simulink model "B2_AutoHeadlamp"  (R2022b)
settings: Solver=FixedStepDiscrete  StartTime=0.0  StopTime=45  FixedStep=Ts  RelTol=1e-3
values from neighbouring files (symbols this model uses):
  LUX_OFF = 2000    [build_B2_AutoHeadlamp.m]
  LUX_ON = 1000    [build_B2_AutoHeadlamp.m]
  T_OFF = 5    [build_B2_AutoHeadlamp.m]
  T_ON = 2    [build_B2_AutoHeadlamp.m]
  T_TUNNEL = 0.3    [build_B2_AutoHeadlamp.m]
  Ts = 0.01    [build_B2_AutoHeadlamp.m]    (also in build_B3_AHB.m)
settings Model: Creator=LENOVO  LastModifiedBy=LENOVO

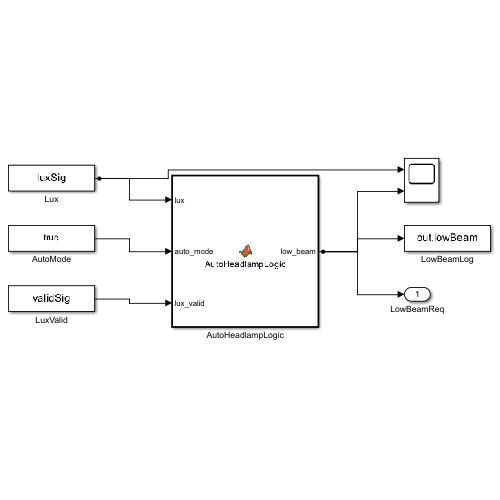
[thumbnail: Simulink's stored preview of the top-level diagram]
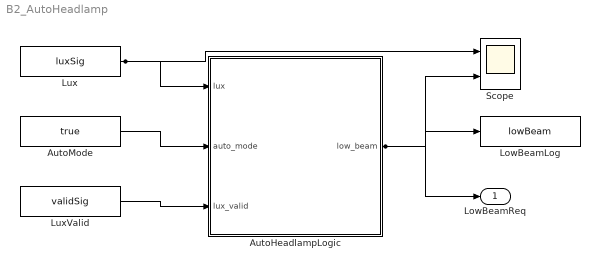
== system B2_AutoHeadlamp ==
  AutoHeadlampLogic : MATLAB Function  TreatAsAtomicUnit=on
  AutoMode : Constant  Value=true  SampleTime=Ts
  LowBeamLog : ToWorkspace  VariableName=lowBeam  SaveFormat=Timeseries  SampleTime=-1
  Lux : FromWorkspace  VariableName=luxSig  SampleTime=Ts  OutputAfterFinalValue=Holding final value
  LuxValid : FromWorkspace  VariableName=validSig  SampleTime=Ts  Interpolate=off  OutputAfterFinalValue=Holding final value
  Scope : Scope  NumInputPorts=2
  LowBeamReq : Outport
  wires:
  Lux/1 -> AutoHeadlampLogic/1(lux), Scope/1
  AutoMode/1 -> AutoHeadlampLogic/2(auto_mode)
  LuxValid/1 -> AutoHeadlampLogic/3(lux_valid)
  AutoHeadlampLogic/1(low_beam) -> LowBeamLog/1, Scope/2, LowBeamReq/1

== matlab function B2_AutoHeadlamp/AutoHeadlampLogic ==
  data: lux input; low_beam output; auto_mode input; lux_valid input; Ts parameter; LUX_ON parameter; LUX_OFF parameter; T_ON parameter; T_OFF parameter; T_TUNNEL parameter
function low_beam = AutoHeadlampLogic(lux, auto_mode, lux_valid, Ts, LUX_ON, LUX_OFF, T_ON, T_OFF, T_TUNNEL)
%#codegen
% B2 - Auto Headlamp : allumage/extinction automatique avec hysteresis
persistent st cnt buf idx
N = 50;                          % 0,5 s d'historique (Ts = 10 ms)
if isempty(st)
    st = false; cnt = 0; buf = 10000*ones(1, N); idx = 1;
end
% Detection tunnel : chute > 80 % en moins de 0,5 s (REQ-LSC-08)
lux_past = buf(idx);
buf(idx) = lux;
idx = mod(idx, N) + 1;
tunnel = (lux < 0.2*lux_past) && (lux < LUX_ON);

if ~auto_mode
    st = false; cnt = 0;
elseif ~lux_valid
    st = true;  cnt = 0;         % etat sur : capteur en defaut (REQ-LSC-09)
elseif ~st
    if lux < LUX_ON
        cnt = cnt + Ts;
        if (cnt > T_ON + Ts/2) || (tunnel && cnt > T_TUNNEL + Ts/2)
            st = true; cnt = 0;
        end
    else
        cnt = 0;
    end
else
    if lux > LUX_OFF
        cnt = cnt + Ts;
        if cnt > T_OFF + Ts/2
            st = false; cnt = 0;
        end
    else
        cnt = 0;
    end
end
low_beam = st;
